simulink model "ACEServoCard"  (R2025b)
settings: Solver=ode4  StartTime=0.0  StopTime=inf  FixedStep=0.01  RelTol=1e-3
undefined symbols (not defined in the file or in its folder): RS422, TTL, UART4, UART5
libraries: simulink x45, etargetslib x26, AFCToolbox x12
settings Model: Creator=zqinghua  LastModifiedBy=zqhkd
settings OptimizationCC: DefaultParameterBehavior=Inlined  EnhancedBackFolding=on  PassReuseOutputArgsAs=Individual arguments  ZeroExternalMemoryAtStartup=off  ZeroInternalMemoryAtStartup=off  OptimizeBlockOrder=speed  DifferentSizesBufferReuse=on  OptimizationCustomize=off  EfficientTunableParamExpr=on
settings DebuggingCC: ParameterTunabilityLossMsg=error
settings HardwareCC: ProdBitPerInt=16.0  ProdBitPerPointer=16.0  ProdBitPerSizeT=16.0  ProdBitPerPtrDiffT=16.0  ProdLargestAtomicFloat=None  ProdWordSize=16.0  ProdHWDeviceType=STMicroelectronics->ST10/Super10
settings SFSimCC: MATLABDynamicMemAlloc=off
settings RTWCC: SystemTargetFile=AFCHawk.tlc  GenCodeOnly=on  TemplateMakefile=ert_default_tmf  GPUComputeCapability=3.5  Description=Embedded Coder
settings CodeAppCC: ForceParamTrailComments=on  IgnoreCustomStorageClasses=off  OperatorAnnotations=on  SimulinkDataObjDesc=on  SFDataObjDesc=on  InsertBlockDesc=on
settings STFCustomTargetCC: SystemTargetFile=AFCHawk.tlc  TargetLangStandard=C99 (ISO)  MultiwordLength=256.0  ModelReferenceCompliant=off  ConcurrentExecutionCompliant=off  CombineOutputUpdateFcns=on  ERTCustomFileBanners=on  SupportContinuousTime=off  SupportNonInlinedSFcns=off  RemoveResetFunc=on  MATLABClassNameForMDSCustomization=Simulink.SoftwareTarget.ERTCustomization  GRTInterface=off  t_DownLoad2Target=on  t_comPort=2.0  t_BuildCPrj2Hex=on  t_comBaud=460800.0
settings ERTTargetCC: ERTCustomFileTemplate=example_file_process.tlc  DynamicArrayContainerType=coder::array  TargetLangStandard=C99 (ISO)  ModelReferenceCompliant=off  ParMdlRefBuildCompliant=off  CompOptLevelCompliant=off  ConcurrentExecutionCompliant=off  ModelStepFunctionPrototypeControlCompliant=off  CPPClassGenCompliant=off  UseToolchainInfoCompliant=off

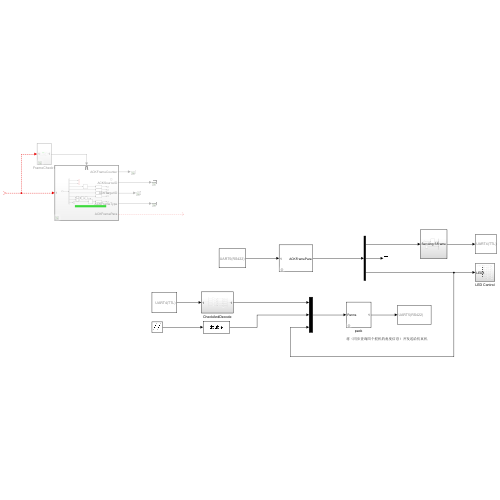
[thumbnail: Simulink's stored preview of the top-level diagram]
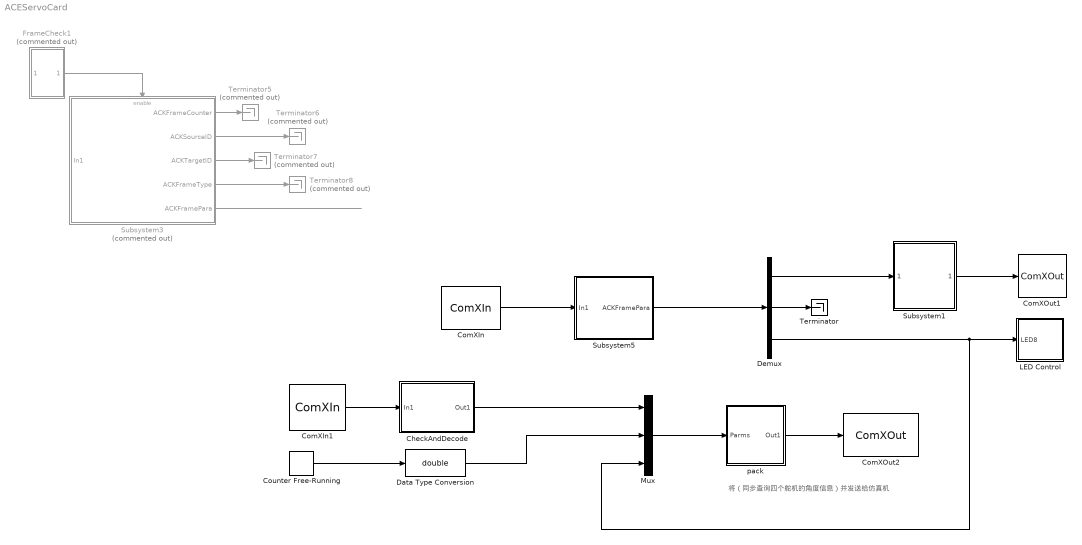
== system ACEServoCard ==
  note: 将（同步查询四个舵机的角度信息）并发送给仿真机
  CheckAndDecode : Subsystem
  ComXIn : AFCToolbox/DeviceModule/ComXIn  Priority=2  g_sampleTime=0.01  g_comPort=UART5(RS422)  g_baudRate=460800  g_dataSize=40  g_parity=0  g_stopBits=1
      settings: SourceProductName=AFCToolbox
  ComXIn1 : AFCToolbox/DeviceModule/ComXIn  Priority=2  g_sampleTime=0.01  g_comPort=UART4(TTL)  g_baudRate=1000000  g_dataSize=4*8  g_parity=0  g_stopBits=1
      settings: SourceProductName=AFCToolbox
  ComXOut1 : AFCToolbox/DeviceModule/ComXOut  Priority=8  g_comPort=UART4(TTL)  g_baudRate=1000000  g_outFreq=1
      settings: SourceProductName=AFCToolbox
  ComXOut2 : AFCToolbox/DeviceModule/ComXOut  Priority=8  g_comPort=UART5(RS422)  g_baudRate=460800  g_outFreq=1
      settings: SourceProductName=AFCToolbox
  Counter Free-Running : simulink/Sources/Counter Free-Running  NumBits=32  tsamp=-1
  Data Type Conversion : DataTypeConversion  OutDataTypeStr=double  SaturateOnIntegerOverflow=off  RndMeth=Floor
  Demux : Demux  Outputs=[4,2,1]
  FrameCheck1 : Subsystem  Commented=on
  LED Control : Subsystem
  Mux : Mux  Inputs=3
  Subsystem1 : Subsystem
  Subsystem3 : Subsystem  Commented=on
  Subsystem5 : Subsystem  mask{length=40, frameType=84}
      mask DialogControl ParameterGroupVar Prompt: 输入字节数
      mask DialogControl Container3 Prompt: 帧类型码(dec)
  Terminator : Terminator
  Terminator{5..8} (4 alike) : Terminator  Commented=on
  pack : Subsystem  mask{frameSender=0, frameType=5}
      mask DialogControl ParameterGroupVar Prompt: 发送方(dec)
      mask DialogControl Container3 Prompt: 帧类型码(dec)
  wires:
  Demux/2 -> Terminator/1
  Demux/1 -> Subsystem1/1(ServAng)
  Demux/3 -> LED Control/1(LED8), Mux/3
  ComXIn1/1 -> CheckAndDecode/1(In1)
  CheckAndDecode/1(Out1) -> Mux/1
  Mux/1 -> pack/1(Parms)
  pack/1(Out1) -> ComXOut2/1
  Subsystem1/1(SFrame) -> ComXOut1/1
  Counter Free-Running/1 -> Data Type Conversion/1
  Data Type Conversion/1 -> Mux/2
  Subsystem3/5(ACKFramePara) -> ?
  ? -> Subsystem3/1(In1), FrameCheck1/1(In1)
  FrameCheck1/1(Out1) -> Subsystem3/Enable
  Subsystem3/4(ACKFrameType) -> Terminator8/1
  Subsystem3/3(ACKTargetID) -> Terminator7/1
  Subsystem3/1(ACKFrameCounter) -> Terminator5/1
  Subsystem3/2(ACKSourceID) -> Terminator6/1
  ComXIn/1 -> Subsystem5/1(In1)
  Subsystem5/1(ACKFramePara) -> Demux/1

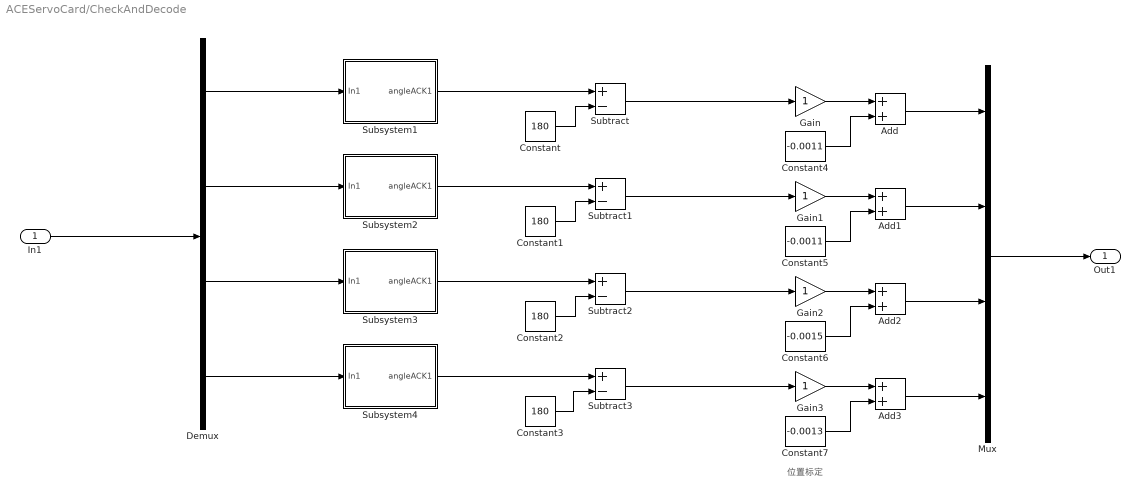
== system ACEServoCard/CheckAndDecode ==
  note: 位置标定
  In1 : Inport
  Add{,1..3} (4 alike) : Sum
  Constant{,1..3} (4 alike) : Constant  Value=180
  Constant4 : Constant  Value=-0.0011
  Constant5 : Constant  Value=-0.0011
  Constant6 : Constant  Value=-0.0015
  Constant7 : Constant  Value=-0.0013
  Demux : Demux  Outputs=[8,8,8,8]
  Gain{,1..3} (4 alike) : Gain
  Mux : Mux
  Subsystem1 : Subsystem
  Subsystem2 : Subsystem
  Subsystem3 : Subsystem
  Subsystem4 : Subsystem
  Subtract{,1..3} (4 alike) : Sum  Inputs=+-
  Out1 : Outport
  wires:
  In1/1 -> Demux/1
  Demux/4 -> Subsystem4/1(In1)
  Demux/3 -> Subsystem3/1(In1)
  Demux/2 -> Subsystem2/1(In1)
  Demux/1 -> Subsystem1/1(In1)
  Subsystem1/1(angleACK1) -> Subtract/1
  Mux/1 -> Out1/1
  Subtract/1 -> Gain/1
  Constant/1 -> Subtract/2
  Constant1/1 -> Subtract1/2
  Subsystem2/1(angleACK1) -> Subtract1/1
  Constant2/1 -> Subtract2/2
  Subsystem3/1(angleACK1) -> Subtract2/1
  Constant3/1 -> Subtract3/2
  Subsystem4/1(angleACK1) -> Subtract3/1
  Constant4/1 -> Add/2
  Gain/1 -> Add/1
  Add/1 -> Mux/1
  Gain1/1 -> Add1/1
  Constant5/1 -> Add1/2
  Subtract1/1 -> Gain1/1
  Subtract2/1 -> Gain2/1
  Constant6/1 -> Add2/2
  Gain2/1 -> Add2/1
  Gain3/1 -> Add3/1
  Constant7/1 -> Add3/2
  Subtract3/1 -> Gain3/1
  Add1/1 -> Mux/2
  Add2/1 -> Mux/3
  Add3/1 -> Mux/4

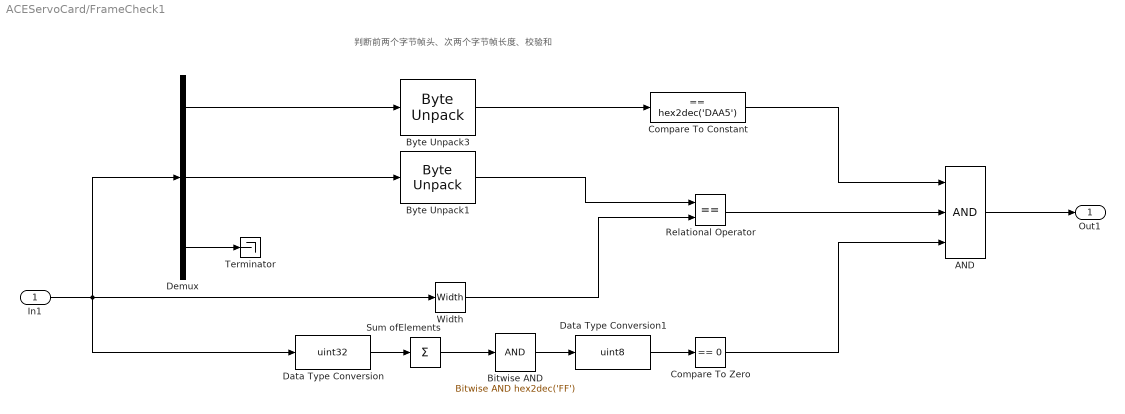
== system ACEServoCard/FrameCheck1 ==
  note: 判断前两个字节帧头、次两个字节帧长度、校验和
  In1 : Inport
  AND : Logic  Inputs=3  IconShape=distinctive  AllPortsSameDT=off  OutDataTypeStr=boolean
  Bitwise AND : simulink/Logic and Bit Operations/Bitwise Operator  logicop=AND  UseBitMask=on  BitMask=hex2dec('FF')  BitMaskRealWorld=Stored Integer
      settings: LibrarySourceBlock=|
      | simulink/Quick Insert/Logic and Bit
      | Operations/Bitwise AND
  Byte Unpack1 : etargetslib/Byte Unpack  dimensions={1}  datatypes={'uint16'}  byteAlign=1
      settings: LibrarySourceBlock=embeddedtargetslib/Host Communication/Byte Unpack
  Byte Unpack3 : etargetslib/Byte Unpack  dimensions={1}  datatypes={'uint16'}  byteAlign=1
      settings: LibrarySourceBlock=embeddedtargetslib/Host Communication/Byte Unpack
  Compare To Constant : simulink/Logic and Bit Operations/Compare To Constant  relop===  const=hex2dec('DAA5')  OutDataTypeStr=boolean
  Compare To Zero : simulink/Logic and Bit Operations/Compare To Zero  relop===  OutDataTypeStr=boolean
  Data Type Conversion : DataTypeConversion  OutDataTypeStr=uint32  SaturateOnIntegerOverflow=off  RndMeth=Floor
  Data Type Conversion1 : DataTypeConversion  OutDataTypeStr=uint8  SaturateOnIntegerOverflow=off  RndMeth=Floor
  Demux : Demux  Outputs=[2,2,-1]
      settings: DisplayOption=none
  Relational Operator : RelationalOperator  Operator===  OutDataTypeStr=boolean  RndMeth=Simplest  InputSameDT=off
  Sum ofElements : Sum  Inputs=+
  Terminator : Terminator
  Width : Width  DataType=uint16
  Out1 : Outport
  wires:
  Sum ofElements/1 -> Bitwise AND/1
  Data Type Conversion1/1 -> Compare To Zero/1
  Demux/3 -> Terminator/1
  Byte Unpack3/1 -> Compare To Constant/1
  Data Type Conversion/1 -> Sum ofElements/1
  In1/1 -> Width/1, Data Type Conversion/1, Demux/1
  Byte Unpack1/1 -> Relational Operator/1
  Demux/2 -> Byte Unpack1/1
  Relational Operator/1 -> AND/2
  Width/1 -> Relational Operator/2
  Compare To Zero/1 -> AND/3
  Compare To Constant/1 -> AND/1
  Demux/1 -> Byte Unpack3/1
  Bitwise AND/1 -> Data Type Conversion1/1
  AND/1 -> Out1/1

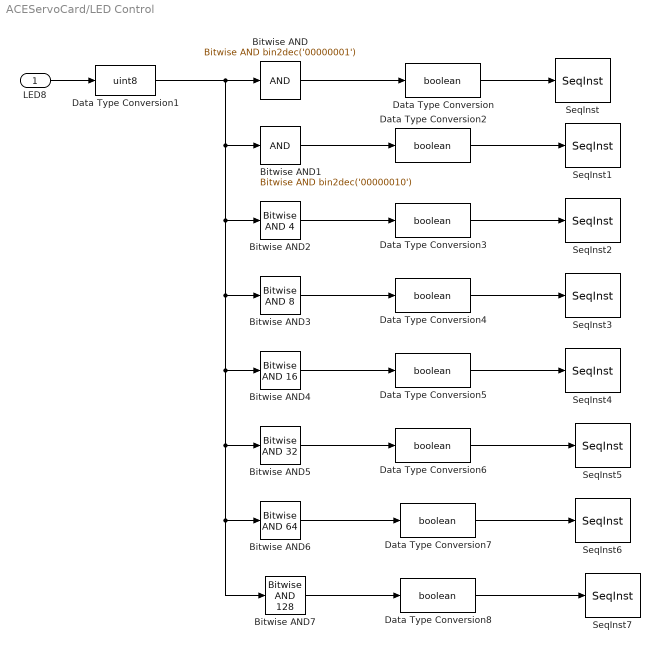
== system ACEServoCard/LED Control ==
  LED8 : Inport
  Bitwise AND : simulink/Logic and Bit Operations/Bitwise Operator  logicop=AND  UseBitMask=on  BitMask=bin2dec('00000001')  BitMaskRealWorld=Stored Integer
      settings: LibrarySourceBlock=|
      | simulink/Quick Insert/Logic and Bit
      | Operations/Bitwise AND
  Bitwise AND1 : simulink/Logic and Bit Operations/Bitwise Operator  logicop=AND  UseBitMask=on  BitMask=bin2dec('00000010')  BitMaskRealWorld=Stored Integer
      settings: LibrarySourceBlock=|
      | simulink/Quick Insert/Logic and Bit
      | Operations/Bitwise AND
  Bitwise AND2 : simulink/Logic and Bit Operations/Bitwise Operator  logicop=AND  UseBitMask=on  BitMask=4  BitMaskRealWorld=Stored Integer
      settings: LibrarySourceBlock=|
      | simulink/Quick Insert/Logic and Bit
      | Operations/Bitwise AND
  Bitwise AND3 : simulink/Logic and Bit Operations/Bitwise Operator  logicop=AND  UseBitMask=on  BitMask=8  BitMaskRealWorld=Stored Integer
      settings: LibrarySourceBlock=|
      | simulink/Quick Insert/Logic and Bit
      | Operations/Bitwise AND
  Bitwise AND4 : simulink/Logic and Bit Operations/Bitwise Operator  logicop=AND  UseBitMask=on  BitMask=16  BitMaskRealWorld=Stored Integer
      settings: LibrarySourceBlock=|
      | simulink/Quick Insert/Logic and Bit
      | Operations/Bitwise AND
  Bitwise AND5 : simulink/Logic and Bit Operations/Bitwise Operator  logicop=AND  UseBitMask=on  BitMask=32  BitMaskRealWorld=Stored Integer
      settings: LibrarySourceBlock=|
      | simulink/Quick Insert/Logic and Bit
      | Operations/Bitwise AND
  Bitwise AND6 : simulink/Logic and Bit Operations/Bitwise Operator  logicop=AND  UseBitMask=on  BitMask=64  BitMaskRealWorld=Stored Integer
      settings: LibrarySourceBlock=|
      | simulink/Quick Insert/Logic and Bit
      | Operations/Bitwise AND
  Bitwise AND7 : simulink/Logic and Bit Operations/Bitwise Operator  logicop=AND  UseBitMask=on  BitMask=128  BitMaskRealWorld=Stored Integer
      settings: LibrarySourceBlock=|
      | simulink/Quick Insert/Logic and Bit
      | Operations/Bitwise AND
  Data Type Conversion{,2..8} (8 alike) : DataTypeConversion  OutDataTypeStr=boolean  SaturateOnIntegerOverflow=off  RndMeth=Floor
  Data Type Conversion1 : DataTypeConversion  OutDataTypeStr=uint8  SaturateOnIntegerOverflow=off  RndMeth=Floor
  SeqInst : AFCToolbox/DeviceModule/SeqInst  Priority=6  g_chanelNo=时序指令1  g_comPort=0  g_instName=0  g_id=0
      settings: SourceProductName=AFCToolbox
  SeqInst1 : AFCToolbox/DeviceModule/SeqInst  Priority=6  g_chanelNo=时序指令2  g_comPort=0  g_instName=0  g_id=0
      settings: SourceProductName=AFCToolbox
  SeqInst2 : AFCToolbox/DeviceModule/SeqInst  Priority=6  g_chanelNo=时序指令3  g_comPort=0  g_instName=0  g_id=0
      settings: SourceProductName=AFCToolbox
  SeqInst3 : AFCToolbox/DeviceModule/SeqInst  Priority=6  g_chanelNo=时序指令4  g_comPort=0  g_instName=0  g_id=0
      settings: SourceProductName=AFCToolbox
  SeqInst4 : AFCToolbox/DeviceModule/SeqInst  Priority=6  g_chanelNo=时序指令5  g_comPort=0  g_instName=0  g_id=0
      settings: SourceProductName=AFCToolbox
  SeqInst5 : AFCToolbox/DeviceModule/SeqInst  Priority=6  g_chanelNo=时序指令6  g_comPort=0  g_instName=0  g_id=0
      settings: SourceProductName=AFCToolbox
  SeqInst6 : AFCToolbox/DeviceModule/SeqInst  Priority=6  g_chanelNo=时序指令7  g_comPort=0  g_instName=0  g_id=0
      settings: SourceProductName=AFCToolbox
  SeqInst7 : AFCToolbox/DeviceModule/SeqInst  Priority=6  g_chanelNo=时序指令8  g_comPort=0  g_instName=0  g_id=0
      settings: SourceProductName=AFCToolbox
  wires:
  Bitwise AND2/1 -> Data Type Conversion3/1
  LED8/1 -> Data Type Conversion1/1
  Bitwise AND5/1 -> Data Type Conversion6/1
  Bitwise AND6/1 -> Data Type Conversion7/1
  Bitwise AND1/1 -> Data Type Conversion2/1
  Bitwise AND3/1 -> Data Type Conversion4/1
  Bitwise AND7/1 -> Data Type Conversion8/1
  Bitwise AND/1 -> Data Type Conversion/1
  Bitwise AND4/1 -> Data Type Conversion5/1
  Data Type Conversion1/1 -> Bitwise AND7/1, Bitwise AND6/1, Bitwise AND5/1, Bitwise AND4/1, Bitwise AND3/1, Bitwise AND2/1, Bitwise AND1/1, Bitwise AND/1
  Data Type Conversion/1 -> SeqInst/1
  Data Type Conversion2/1 -> SeqInst1/1
  Data Type Conversion3/1 -> SeqInst2/1
  Data Type Conversion4/1 -> SeqInst3/1
  Data Type Conversion5/1 -> SeqInst4/1
  Data Type Conversion6/1 -> SeqInst5/1
  Data Type Conversion7/1 -> SeqInst6/1
  Data Type Conversion8/1 -> SeqInst7/1

== system ACEServoCard/Subsystem1 ==
  ServAng : Inport
  Mux : Mux  Inputs=2
  查询四个舵机角度指令 : Subsystem
  设置四个舵机位置与速度指令 : Subsystem
  SFrame : Outport
  wires:
  查询四个舵机角度指令/1(RAng) -> Mux/2
  Mux/1 -> SFrame/1
  设置四个舵机位置与速度指令/1(Frame) -> Mux/1
  ServAng/1 -> 设置四个舵机位置与速度指令/1(Ang)

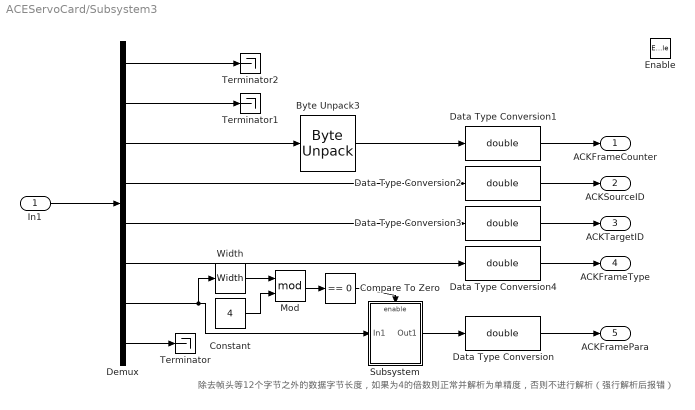
== system ACEServoCard/Subsystem3 ==
  note: 除去帧头等12个字节之外的数据字节长度，如果为4的倍数则正常并解析为单精度，否则不进行解析（强行解析后报错）
  In1 : Inport
  Enable : EnablePort
  Byte Unpack3 : etargetslib/Byte Unpack  dimensions={1}  datatypes={'uint32'}  byteAlign=1
      settings: LibrarySourceBlock=embeddedtargetslib/Host Communication/Byte Unpack
  Compare To Zero : simulink/Logic and Bit Operations/Compare To Zero  relop===  OutDataTypeStr=boolean
  Constant : Constant  Value=4  OutDataTypeStr=uint16
  Data Type Conversion{,1..4} (5 alike) : DataTypeConversion  OutDataTypeStr=double  SaturateOnIntegerOverflow=off  RndMeth=Floor
  Demux : Demux  Outputs=[2,2,4,1,1,1,-1,1]
      settings: DisplayOption=none
  Mod : Math  Operator=mod
  Subsystem : Subsystem
  Terminator : Terminator
  Terminator1 : Terminator
  Terminator2 : Terminator
  Width : Width  DataType=uint16
  ACKFrameCounter : Outport
  ACKSourceID : Outport  Port=2
  ACKTargetID : Outport  Port=3
  ACKFrameType : Outport  Port=4
  ACKFramePara : Outport  Port=5
  wires:
  Compare To Zero/1 -> Subsystem/Enable
  Mod/1 -> Compare To Zero/1
  Data Type Conversion/1 -> ACKFramePara/1
  Subsystem/1(Out1) -> Data Type Conversion/1
  Demux/1 -> Terminator2/1
  Data Type Conversion2/1 -> ACKSourceID/1
  Demux/7 -> Width/1, Subsystem/1(In1)
  Demux/2 -> Terminator1/1
  Demux/5 -> Data Type Conversion3/1
  Demux/6 -> Data Type Conversion4/1
  Data Type Conversion1/1 -> ACKFrameCounter/1
  Data Type Conversion4/1 -> ACKFrameType/1
  Demux/3 -> Byte Unpack3/1
  Byte Unpack3/1 -> Data Type Conversion1/1
  Width/1 -> Mod/1
  Demux/8 -> Terminator/1
  In1/1 -> Demux/1
  Demux/4 -> Data Type Conversion2/1
  Data Type Conversion3/1 -> ACKTargetID/1
  Constant/1 -> Mod/2

== system ACEServoCard/Subsystem5 ==
  In1 : Inport
  FrameCheck1 : Subsystem
  Subsystem1 : Subsystem
  Terminator{1..4} (4 alike) : Terminator
  ACKFramePara : Outport
  wires:
  Subsystem1/4(ACKFrameType) -> Terminator4/1
  Subsystem1/2(ACKSourceID) -> Terminator2/1
  In1/1 -> Subsystem1/1(In1), FrameCheck1/1(In1)
  Subsystem1/1(ACKFrameCounter) -> Terminator1/1  "AFC_ACK_COUNTER"
  FrameCheck1/1(Out1) -> Subsystem1/Enable
  Subsystem1/3(ACKTargetID) -> Terminator3/1
  Subsystem1/5(ACKFramePara) -> ACKFramePara/1

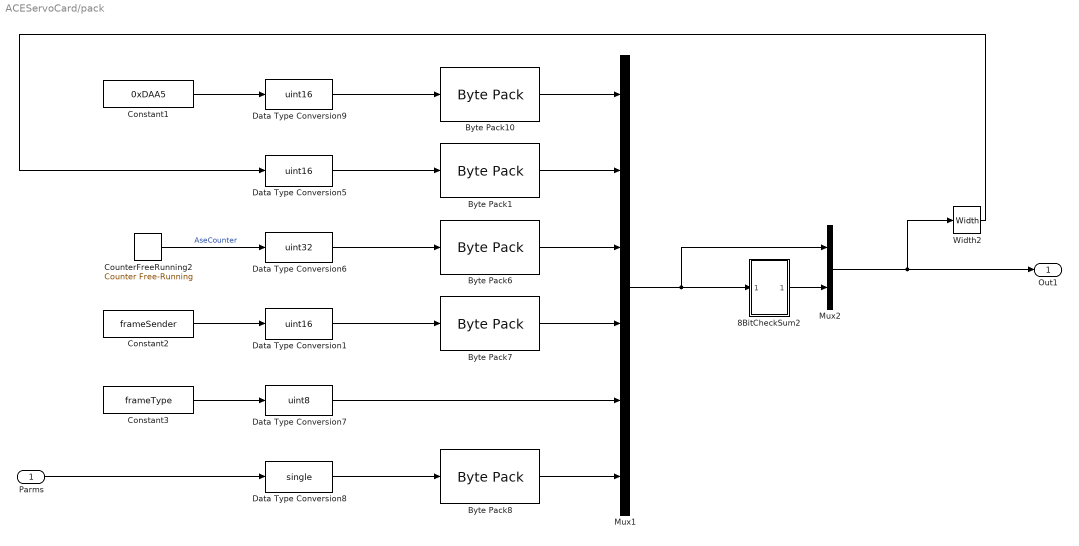
== system ACEServoCard/pack ==
  Parms : Inport
  8BitCheckSum2 : Subsystem
  Byte Pack1 : etargetslib/Byte Pack  datatypes={'uint16'}  byteAlign=1
  Byte Pack10 : etargetslib/Byte Pack  datatypes={'uint16'}  byteAlign=1
  Byte Pack6 : etargetslib/Byte Pack  datatypes={'uint32'}  byteAlign=1
  Byte Pack7 : etargetslib/Byte Pack  datatypes={'uint16'}  byteAlign=1
  Byte Pack8 : etargetslib/Byte Pack  datatypes={'single'}  byteAlign=1
  Constant1 : Constant  Value=0xDAA5
  Constant2 : Constant  Value=frameSender
  Constant3 : Constant  Value=frameType
  CounterFreeRunning2 : simulink/Sources/Counter Free-Running  NumBits=32  tsamp=-1
  Data Type Conversion1 : DataTypeConversion  OutDataTypeStr=uint16  SaturateOnIntegerOverflow=off  RndMeth=Floor
  Data Type Conversion5 : DataTypeConversion  OutDataTypeStr=uint16  SaturateOnIntegerOverflow=off  RndMeth=Floor
  Data Type Conversion6 : DataTypeConversion  OutDataTypeStr=uint32  SaturateOnIntegerOverflow=off  RndMeth=Floor
  Data Type Conversion7 : DataTypeConversion  OutDataTypeStr=uint8  SaturateOnIntegerOverflow=off  RndMeth=Floor
  Data Type Conversion8 : DataTypeConversion  OutDataTypeStr=single  SaturateOnIntegerOverflow=off  RndMeth=Floor
  Data Type Conversion9 : DataTypeConversion  OutDataTypeStr=uint16  SaturateOnIntegerOverflow=off  RndMeth=Floor
  Mux1 : Mux  Inputs=6
  Mux2 : Mux  Inputs=2
  Width2 : Width  DataType=single
  Out1 : Outport
  wires:
  Data Type Conversion6/1 -> Byte Pack6/1
  Data Type Conversion9/1 -> Byte Pack10/1
  Byte Pack6/1 -> Mux1/3
  Mux1/1 -> Mux2/1, 8BitCheckSum2/1(In1)
  Byte Pack8/1 -> Mux1/6
  Data Type Conversion8/1 -> Byte Pack8/1
  8BitCheckSum2/1(Out1) -> Mux2/2
  Byte Pack1/1 -> Mux1/2
  Data Type Conversion1/1 -> Byte Pack7/1
  Byte Pack7/1 -> Mux1/4
  Width2/1 -> Data Type Conversion5/1
  Constant2/1 -> Data Type Conversion1/1
  Byte Pack10/1 -> Mux1/1
  Data Type Conversion7/1 -> Mux1/5
  Constant1/1 -> Data Type Conversion9/1
  CounterFreeRunning2/1 -> Data Type Conversion6/1  "AseCounter"
  Constant3/1 -> Data Type Conversion7/1
  Data Type Conversion5/1 -> Byte Pack1/1
  Parms/1 -> Data Type Conversion8/1
  Mux2/1 -> Out1/1, Width2/1

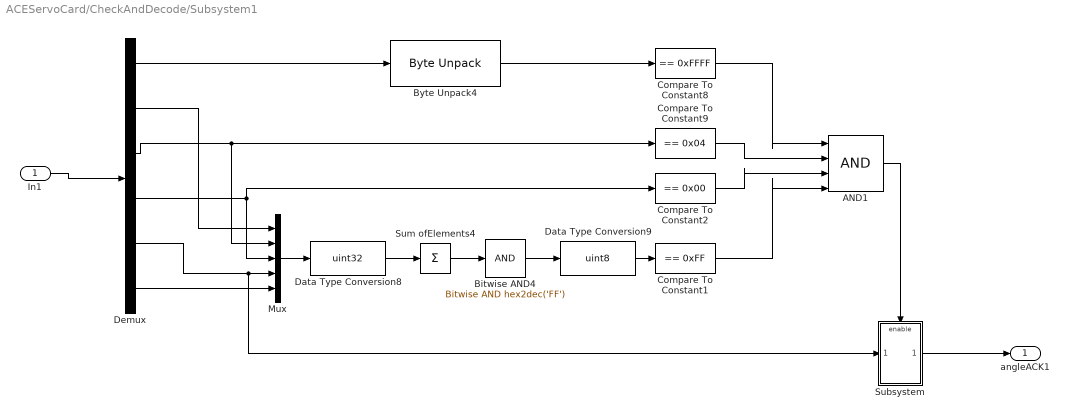
== system ACEServoCard/CheckAndDecode/Subsystem1 ==
  In1 : Inport
  AND1 : Logic  Inputs=4  IconShape=distinctive  AllPortsSameDT=off  OutDataTypeStr=boolean
  Bitwise AND4 : simulink/Logic and Bit Operations/Bitwise Operator  logicop=AND  UseBitMask=on  BitMask=hex2dec('FF')  BitMaskRealWorld=Stored Integer
      settings: LibrarySourceBlock=|
      | simulink/Quick Insert/Logic and Bit
      | Operations/Bitwise AND
  Byte Unpack4 : etargetslib/Byte Unpack  dimensions={[1]}  datatypes={'uint16'}  byteAlign=1
      settings: LibrarySourceBlock=embeddedtargetslib/Host Communication/Byte Unpack
  Compare To Constant1 : simulink/Logic and Bit Operations/Compare To Constant  relop===  const=0xFF  OutDataTypeStr=boolean
  Compare To Constant2 : simulink/Logic and Bit Operations/Compare To Constant  relop===  const=0x00  OutDataTypeStr=boolean
  Compare To Constant8 : simulink/Logic and Bit Operations/Compare To Constant  relop===  const=0xFFFF  OutDataTypeStr=boolean
  Compare To Constant9 : simulink/Logic and Bit Operations/Compare To Constant  relop===  const=0x04  OutDataTypeStr=boolean
  Data Type Conversion8 : DataTypeConversion  OutDataTypeStr=uint32  SaturateOnIntegerOverflow=off  RndMeth=Floor
  Data Type Conversion9 : DataTypeConversion  OutDataTypeStr=uint8  SaturateOnIntegerOverflow=off  RndMeth=Floor
  Demux : Demux  Outputs=[2,1,1,1,2,1]
  Mux : Mux  Inputs=5
  Subsystem : Subsystem
  Sum ofElements4 : Sum  Inputs=+
  angleACK1 : Outport
  wires:
  AND1/1 -> Subsystem/Enable
  Demux/6 -> Mux/5
  Subsystem/1(Outport) -> angleACK1/1
  Demux/5 -> Subsystem/1(In1), Mux/4
  Demux/3 -> Mux/2, Compare To Constant9/1
  Compare To Constant2/1 -> AND1/3
  Demux/2 -> Mux/1
  Data Type Conversion8/1 -> Sum ofElements4/1
  Compare To Constant9/1 -> AND1/2
  Sum ofElements4/1 -> Bitwise AND4/1
  Demux/4 -> Compare To Constant2/1, Mux/3
  Byte Unpack4/1 -> Compare To Constant8/1
  Mux/1 -> Data Type Conversion8/1
  Compare To Constant8/1 -> AND1/1
  Data Type Conversion9/1 -> Compare To Constant1/1
  Bitwise AND4/1 -> Data Type Conversion9/1
  Demux/1 -> Byte Unpack4/1
  Compare To Constant1/1 -> AND1/4
  In1/1 -> Demux/1

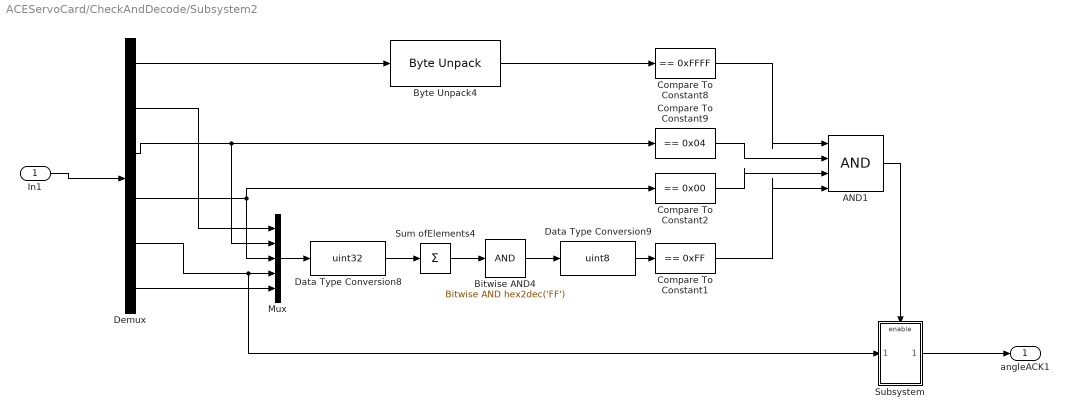
== system ACEServoCard/CheckAndDecode/Subsystem2 ==
  In1 : Inport
  AND1 : Logic  Inputs=4  IconShape=distinctive  AllPortsSameDT=off  OutDataTypeStr=boolean
  Bitwise AND4 : simulink/Logic and Bit Operations/Bitwise Operator  logicop=AND  UseBitMask=on  BitMask=hex2dec('FF')  BitMaskRealWorld=Stored Integer
      settings: LibrarySourceBlock=|
      | simulink/Quick Insert/Logic and Bit
      | Operations/Bitwise AND
  Byte Unpack4 : etargetslib/Byte Unpack  dimensions={[1]}  datatypes={'uint16'}  byteAlign=1
      settings: LibrarySourceBlock=embeddedtargetslib/Host Communication/Byte Unpack
  Compare To Constant1 : simulink/Logic and Bit Operations/Compare To Constant  relop===  const=0xFF  OutDataTypeStr=boolean
  Compare To Constant2 : simulink/Logic and Bit Operations/Compare To Constant  relop===  const=0x00  OutDataTypeStr=boolean
  Compare To Constant8 : simulink/Logic and Bit Operations/Compare To Constant  relop===  const=0xFFFF  OutDataTypeStr=boolean
  Compare To Constant9 : simulink/Logic and Bit Operations/Compare To Constant  relop===  const=0x04  OutDataTypeStr=boolean
  Data Type Conversion8 : DataTypeConversion  OutDataTypeStr=uint32  SaturateOnIntegerOverflow=off  RndMeth=Floor
  Data Type Conversion9 : DataTypeConversion  OutDataTypeStr=uint8  SaturateOnIntegerOverflow=off  RndMeth=Floor
  Demux : Demux  Outputs=[2,1,1,1,2,1]
  Mux : Mux  Inputs=5
  Subsystem : Subsystem
  Sum ofElements4 : Sum  Inputs=+
  angleACK1 : Outport
  wires:
  In1/1 -> Demux/1
  Compare To Constant1/1 -> AND1/4
  Demux/1 -> Byte Unpack4/1
  Bitwise AND4/1 -> Data Type Conversion9/1
  Data Type Conversion9/1 -> Compare To Constant1/1
  Compare To Constant8/1 -> AND1/1
  Mux/1 -> Data Type Conversion8/1
  Byte Unpack4/1 -> Compare To Constant8/1
  Demux/4 -> Mux/3, Compare To Constant2/1
  Sum ofElements4/1 -> Bitwise AND4/1
  Compare To Constant9/1 -> AND1/2
  Data Type Conversion8/1 -> Sum ofElements4/1
  Demux/2 -> Mux/1
  Compare To Constant2/1 -> AND1/3
  Demux/3 -> Compare To Constant9/1, Mux/2
  Demux/5 -> Mux/4, Subsystem/1(In1)
  Subsystem/1(Outport) -> angleACK1/1
  Demux/6 -> Mux/5
  AND1/1 -> Subsystem/Enable

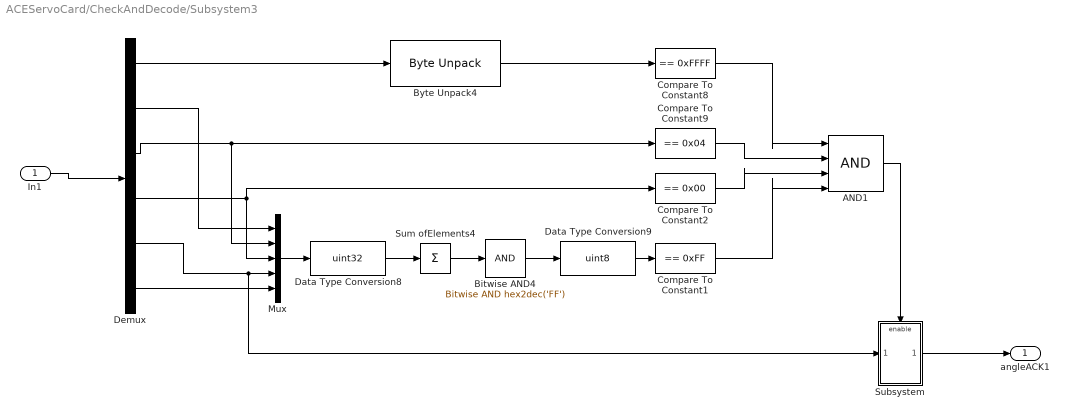
== system ACEServoCard/CheckAndDecode/Subsystem3 ==
  In1 : Inport
  AND1 : Logic  Inputs=4  IconShape=distinctive  AllPortsSameDT=off  OutDataTypeStr=boolean
  Bitwise AND4 : simulink/Logic and Bit Operations/Bitwise Operator  logicop=AND  UseBitMask=on  BitMask=hex2dec('FF')  BitMaskRealWorld=Stored Integer
      settings: LibrarySourceBlock=|
      | simulink/Quick Insert/Logic and Bit
      | Operations/Bitwise AND
  Byte Unpack4 : etargetslib/Byte Unpack  dimensions={[1]}  datatypes={'uint16'}  byteAlign=1
      settings: LibrarySourceBlock=embeddedtargetslib/Host Communication/Byte Unpack
  Compare To Constant1 : simulink/Logic and Bit Operations/Compare To Constant  relop===  const=0xFF  OutDataTypeStr=boolean
  Compare To Constant2 : simulink/Logic and Bit Operations/Compare To Constant  relop===  const=0x00  OutDataTypeStr=boolean
  Compare To Constant8 : simulink/Logic and Bit Operations/Compare To Constant  relop===  const=0xFFFF  OutDataTypeStr=boolean
  Compare To Constant9 : simulink/Logic and Bit Operations/Compare To Constant  relop===  const=0x04  OutDataTypeStr=boolean
  Data Type Conversion8 : DataTypeConversion  OutDataTypeStr=uint32  SaturateOnIntegerOverflow=off  RndMeth=Floor
  Data Type Conversion9 : DataTypeConversion  OutDataTypeStr=uint8  SaturateOnIntegerOverflow=off  RndMeth=Floor
  Demux : Demux  Outputs=[2,1,1,1,2,1]
  Mux : Mux  Inputs=5
  Subsystem : Subsystem
  Sum ofElements4 : Sum  Inputs=+
  angleACK1 : Outport
  wires:
  AND1/1 -> Subsystem/Enable
  Demux/6 -> Mux/5
  Subsystem/1(Outport) -> angleACK1/1
  Demux/5 -> Subsystem/1(In1), Mux/4
  Demux/3 -> Mux/2, Compare To Constant9/1
  Compare To Constant2/1 -> AND1/3
  Demux/2 -> Mux/1
  Data Type Conversion8/1 -> Sum ofElements4/1
  Compare To Constant9/1 -> AND1/2
  Sum ofElements4/1 -> Bitwise AND4/1
  Demux/4 -> Compare To Constant2/1, Mux/3
  Byte Unpack4/1 -> Compare To Constant8/1
  Mux/1 -> Data Type Conversion8/1
  Compare To Constant8/1 -> AND1/1
  Data Type Conversion9/1 -> Compare To Constant1/1
  Bitwise AND4/1 -> Data Type Conversion9/1
  Demux/1 -> Byte Unpack4/1
  Compare To Constant1/1 -> AND1/4
  In1/1 -> Demux/1

== system ACEServoCard/CheckAndDecode/Subsystem4 ==
  In1 : Inport
  AND1 : Logic  Inputs=4  IconShape=distinctive  AllPortsSameDT=off  OutDataTypeStr=boolean
  Bitwise AND4 : simulink/Logic and Bit Operations/Bitwise Operator  logicop=AND  UseBitMask=on  BitMask=hex2dec('FF')  BitMaskRealWorld=Stored Integer
      settings: LibrarySourceBlock=|
      | simulink/Quick Insert/Logic and Bit
      | Operations/Bitwise AND
  Byte Unpack4 : etargetslib/Byte Unpack  dimensions={[1]}  datatypes={'uint16'}  byteAlign=1
      settings: LibrarySourceBlock=embeddedtargetslib/Host Communication/Byte Unpack
  Compare To Constant1 : simulink/Logic and Bit Operations/Compare To Constant  relop===  const=0xFF  OutDataTypeStr=boolean
  Compare To Constant2 : simulink/Logic and Bit Operations/Compare To Constant  relop===  const=0x00  OutDataTypeStr=boolean
  Compare To Constant8 : simulink/Logic and Bit Operations/Compare To Constant  relop===  const=0xFFFF  OutDataTypeStr=boolean
  Compare To Constant9 : simulink/Logic and Bit Operations/Compare To Constant  relop===  const=0x04  OutDataTypeStr=boolean
  Data Type Conversion8 : DataTypeConversion  OutDataTypeStr=uint32  SaturateOnIntegerOverflow=off  RndMeth=Floor
  Data Type Conversion9 : DataTypeConversion  OutDataTypeStr=uint8  SaturateOnIntegerOverflow=off  RndMeth=Floor
  Demux : Demux  Outputs=[2,1,1,1,2,1]
  Mux : Mux  Inputs=5
  Subsystem : Subsystem
  Sum ofElements4 : Sum  Inputs=+
  angleACK1 : Outport
  wires:
  In1/1 -> Demux/1
  Compare To Constant1/1 -> AND1/4
  Demux/1 -> Byte Unpack4/1
  Bitwise AND4/1 -> Data Type Conversion9/1
  Data Type Conversion9/1 -> Compare To Constant1/1
  Compare To Constant8/1 -> AND1/1
  Mux/1 -> Data Type Conversion8/1
  Byte Unpack4/1 -> Compare To Constant8/1
  Demux/4 -> Mux/3, Compare To Constant2/1
  Sum ofElements4/1 -> Bitwise AND4/1
  Compare To Constant9/1 -> AND1/2
  Data Type Conversion8/1 -> Sum ofElements4/1
  Demux/2 -> Mux/1
  Compare To Constant2/1 -> AND1/3
  Demux/3 -> Compare To Constant9/1, Mux/2
  Demux/5 -> Mux/4, Subsystem/1(In1)
  Subsystem/1(Outport) -> angleACK1/1
  Demux/6 -> Mux/5
  AND1/1 -> Subsystem/Enable

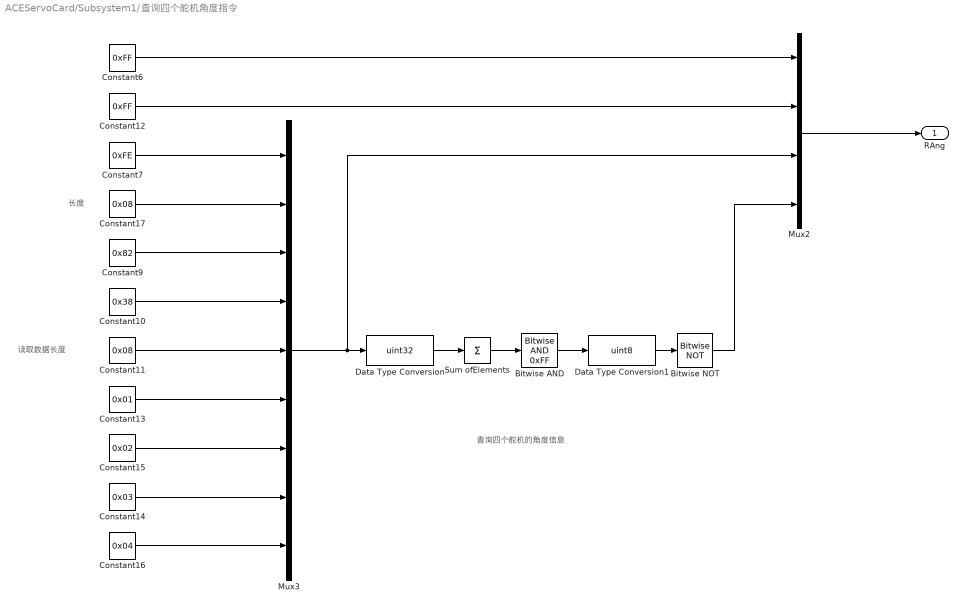
== system ACEServoCard/Subsystem1/查询四个舵机角度指令 ==
  note: 查询四个舵机的角度信息
  note: 长度
  note: 读取数据长度
  Bitwise AND : simulink/Logic and Bit Operations/Bitwise Operator  logicop=AND  UseBitMask=on  BitMask=0xFF  BitMaskRealWorld=Stored Integer
      settings: LibrarySourceBlock=|
      | simulink/Quick Insert/Logic and Bit
      | Operations/Bitwise AND
  Bitwise NOT : simulink/Logic and Bit Operations/Bitwise Operator  logicop=NOT  UseBitMask=off  BitMask=bin2dec('11011001')  BitMaskRealWorld=Stored Integer
      settings: LibrarySourceBlock=|
      | simulink/Quick Insert/Logic and Bit
      | Operations/Bitwise NOT
  Constant10 : Constant  Value=0x38  OutDataTypeStr=uint8
  Constant11 : Constant  Value=0x08  OutDataTypeStr=uint8
  Constant12 : Constant  Value=0xFF  OutDataTypeStr=uint8
  Constant13 : Constant  Value=0x01
  Constant14 : Constant  Value=0x03
  Constant15 : Constant  Value=0x02
  Constant16 : Constant  Value=0x04
  Constant17 : Constant  Value=0x08  OutDataTypeStr=uint8
  Constant6 : Constant  Value=0xFF  OutDataTypeStr=uint8
  Constant7 : Constant  Value=0xFE  OutDataTypeStr=uint8
  Constant9 : Constant  Value=0x82  OutDataTypeStr=uint8
  Data Type Conversion : DataTypeConversion  OutDataTypeStr=uint32  SaturateOnIntegerOverflow=off  RndMeth=Floor
  Data Type Conversion1 : DataTypeConversion  OutDataTypeStr=uint8  SaturateOnIntegerOverflow=off  RndMeth=Floor
  Mux2 : Mux
  Mux3 : Mux  Inputs=9
  Sum ofElements : Sum  Inputs=+
  RAng : Outport
  wires:
  Constant16/1 -> Mux3/9
  Mux3/1 -> Data Type Conversion/1, Mux2/3
  Bitwise AND/1 -> Data Type Conversion1/1
  Data Type Conversion1/1 -> Bitwise NOT/1
  Constant17/1 -> Mux3/2
  Mux2/1 -> RAng/1
  Constant12/1 -> Mux2/2
  Data Type Conversion/1 -> Sum ofElements/1
  Sum ofElements/1 -> Bitwise AND/1
  Constant14/1 -> Mux3/8
  Constant6/1 -> Mux2/1
  Constant13/1 -> Mux3/6
  Constant15/1 -> Mux3/7
  Constant10/1 -> Mux3/4
  Constant11/1 -> Mux3/5
  Bitwise NOT/1 -> Mux2/4
  Constant7/1 -> Mux3/1
  Constant9/1 -> Mux3/3

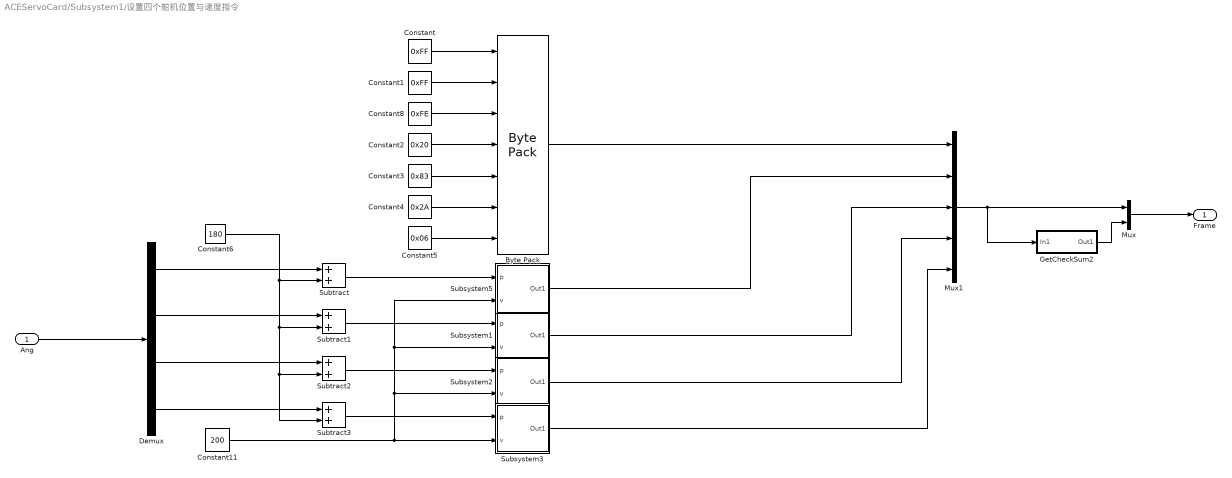
== system ACEServoCard/Subsystem1/设置四个舵机位置与速度指令 ==
  Ang : Inport
  Byte Pack : etargetslib/Byte Pack  datatypes={'uint8','uint8','uint8','uint8','uint8','uint8','uint8'}  byteAlign=1
  Constant : Constant  Value=0xFF  OutDataTypeStr=uint8
  Constant1 : Constant  Value=0xFF  OutDataTypeStr=uint8
  Constant11 : Constant  Value=200
  Constant2 : Constant  Value=0x20  OutDataTypeStr=uint8
  Constant3 : Constant  Value=0x83  OutDataTypeStr=uint8
  Constant4 : Constant  Value=0x2A  OutDataTypeStr=uint8
  Constant5 : Constant  Value=0x06  OutDataTypeStr=uint8
  Constant6 : Constant  Value=180
  Constant8 : Constant  Value=0xFE  OutDataTypeStr=uint8
  Demux : Demux
  GetCheckSum2 : Subsystem
  Mux : Mux  Inputs=2
  Mux1 : Mux  Inputs=5
  Subsystem1 : Subsystem  mask{id=2}
      mask DialogControl ParameterGroupVar Prompt: id
  Subsystem2 : Subsystem  mask{id=3}
      mask DialogControl ParameterGroupVar Prompt: id
  Subsystem3 : Subsystem  mask{id=4}
      mask DialogControl ParameterGroupVar Prompt: id
  Subsystem5 : Subsystem  mask{id=1}
      mask DialogControl ParameterGroupVar Prompt: id
  Subtract{,1..3} (4 alike) : Sum
  Frame : Outport
  wires:
  Mux/1 -> Frame/1
  Constant4/1 -> Byte Pack/6
  Mux1/1 -> Mux/1, GetCheckSum2/1(In1)
  GetCheckSum2/1(Out1) -> Mux/2
  Constant5/1 -> Byte Pack/7
  Constant2/1 -> Byte Pack/4
  Constant1/1 -> Byte Pack/2
  Constant/1 -> Byte Pack/1
  Constant3/1 -> Byte Pack/5
  Constant8/1 -> Byte Pack/3
  Byte Pack/1 -> Mux1/1
  Demux/3 -> Subtract2/1
  Subtract2/1 -> Subsystem2/1(p)
  Subtract3/1 -> Subsystem3/1(p)
  Ang/1 -> Demux/1
  Demux/1 -> Subtract/1
  Constant6/1 -> Subtract3/2, Subtract2/2, Subtract1/2, Subtract/2
  Constant11/1 -> Subsystem3/2(v), Subsystem5/2(v), Subsystem1/2(v), Subsystem2/2(v)
  Subtract1/1 -> Subsystem1/1(p)
  Subtract/1 -> Subsystem5/1(p)
  Demux/2 -> Subtract1/1
  Demux/4 -> Subtract3/1
  Subsystem5/1(Out1) -> Mux1/2
  Subsystem1/1(Out1) -> Mux1/3
  Subsystem2/1(Out1) -> Mux1/4
  Subsystem3/1(Out1) -> Mux1/5

== system ACEServoCard/Subsystem3/Subsystem ==
  In1 : Inport
  Enable : EnablePort
  Byte Unpack1 : etargetslib/Byte Unpack  dimensions={7}  datatypes={'single'}  byteAlign=1
      settings: LibrarySourceBlock=embeddedtargetslib/Host Communication/Byte Unpack
  Out1 : Outport
  wires:
  In1/1 -> Byte Unpack1/1
  Byte Unpack1/1 -> Out1/1

== system ACEServoCard/Subsystem5/FrameCheck1 ==
  note: 判断前两个字节帧头、次1个字节帧长度、校验和
  In1 : Inport
  AND : Logic  Inputs=3  IconShape=distinctive  AllPortsSameDT=off  OutDataTypeStr=boolean
  Bitwise AND : simulink/Logic and Bit Operations/Bitwise Operator  logicop=AND  UseBitMask=on  BitMask=hex2dec('FF')  BitMaskRealWorld=Stored Integer
      settings: LibrarySourceBlock=|
      | simulink/Quick Insert/Logic and Bit
      | Operations/Bitwise AND
  Byte Unpack1 : etargetslib/Byte Unpack  dimensions={1}  datatypes={'uint16'}  byteAlign=1
      settings: LibrarySourceBlock=embeddedtargetslib/Host Communication/Byte Unpack
  Byte Unpack3 : etargetslib/Byte Unpack  dimensions={1}  datatypes={'uint16'}  byteAlign=1
      settings: LibrarySourceBlock=embeddedtargetslib/Host Communication/Byte Unpack
  Compare To Constant : simulink/Logic and Bit Operations/Compare To Constant  relop===  const=0xDAA5  OutDataTypeStr=boolean
  Compare To Zero : simulink/Logic and Bit Operations/Compare To Zero  relop===  OutDataTypeStr=boolean
  Data Type Conversion : DataTypeConversion  OutDataTypeStr=uint32  SaturateOnIntegerOverflow=off  RndMeth=Floor
  Data Type Conversion1 : DataTypeConversion  OutDataTypeStr=uint8  SaturateOnIntegerOverflow=off  RndMeth=Floor
  Demux : Demux  Outputs=[2,2,-1]
      settings: DisplayOption=none
  Relational Operator : RelationalOperator  Operator===  OutDataTypeStr=boolean  RndMeth=Simplest  InputSameDT=off
  Sum ofElements : Sum  Inputs=+
  Terminator : Terminator
  Width : Width  DataType=uint16
  Out1 : Outport
  wires:
  Byte Unpack1/1 -> Relational Operator/1
  Sum ofElements/1 -> Bitwise AND/1
  Data Type Conversion1/1 -> Compare To Zero/1
  Demux/3 -> Terminator/1
  Byte Unpack3/1 -> Compare To Constant/1
  Data Type Conversion/1 -> Sum ofElements/1
  In1/1 -> Width/1, Data Type Conversion/1, Demux/1
  Demux/2 -> Byte Unpack1/1
  Relational Operator/1 -> AND/2
  Width/1 -> Relational Operator/2
  Compare To Zero/1 -> AND/3
  Compare To Constant/1 -> AND/1
  Demux/1 -> Byte Unpack3/1
  Bitwise AND/1 -> Data Type Conversion1/1
  AND/1 -> Out1/1

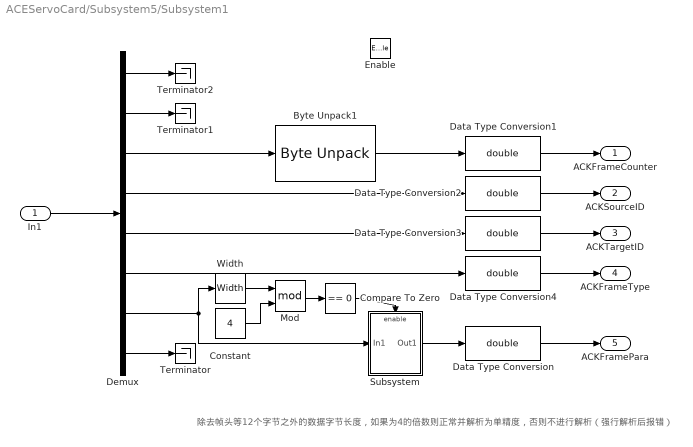
== system ACEServoCard/Subsystem5/Subsystem1 ==
  note: 除去帧头等12个字节之外的数据字节长度，如果为4的倍数则正常并解析为单精度，否则不进行解析（强行解析后报错）
  In1 : Inport
  Enable : EnablePort
  Byte Unpack1 : etargetslib/Byte Unpack  dimensions={1}  datatypes={'uint32'}  byteAlign=1
      settings: LibrarySourceBlock=embeddedtargetslib/Host Communication/Byte Unpack
  Compare To Zero : simulink/Logic and Bit Operations/Compare To Zero  relop===  OutDataTypeStr=boolean
  Constant : Constant  Value=4  OutDataTypeStr=uint16
  Data Type Conversion{,1..4} (5 alike) : DataTypeConversion  OutDataTypeStr=double  SaturateOnIntegerOverflow=off  RndMeth=Floor
  Demux : Demux  Outputs=[2,2,4,1,1,1,-1,1]
      settings: DisplayOption=none
  Mod : Math  Operator=mod
  Subsystem : Subsystem
  Terminator : Terminator
  Terminator1 : Terminator
  Terminator2 : Terminator
  Width : Width  DataType=uint16
  ACKFrameCounter : Outport
  ACKSourceID : Outport  Port=2
  ACKTargetID : Outport  Port=3
  ACKFrameType : Outport  Port=4
  ACKFramePara : Outport  Port=5
  wires:
  Byte Unpack1/1 -> Data Type Conversion1/1
  Compare To Zero/1 -> Subsystem/Enable
  Mod/1 -> Compare To Zero/1
  Data Type Conversion/1 -> ACKFramePara/1
  Demux/1 -> Terminator2/1
  Data Type Conversion2/1 -> ACKSourceID/1
  Demux/7 -> Width/1, Subsystem/1(In1)
  Demux/2 -> Terminator1/1
  Demux/5 -> Data Type Conversion3/1
  Demux/6 -> Data Type Conversion4/1
  Data Type Conversion1/1 -> ACKFrameCounter/1
  Data Type Conversion4/1 -> ACKFrameType/1
  Demux/3 -> Byte Unpack1/1
  Width/1 -> Mod/1
  Demux/8 -> Terminator/1
  In1/1 -> Demux/1
  Demux/4 -> Data Type Conversion2/1
  Data Type Conversion3/1 -> ACKTargetID/1
  Constant/1 -> Mod/2
  Subsystem/1(Out1) -> Data Type Conversion/1

== system ACEServoCard/pack/8BitCheckSum2 ==
  In1 : Inport
  Add : Sum
  Bitwise AND : simulink/Logic and Bit Operations/Bitwise Operator  logicop=AND  UseBitMask=on  BitMask=hex2dec('FF')  BitMaskRealWorld=Stored Integer
      settings: LibrarySourceBlock=|
      | simulink/Quick Insert/Logic and Bit
      | Operations/Bitwise AND
  Bitwise AND1 : simulink/Logic and Bit Operations/Bitwise Operator  logicop=AND  UseBitMask=on  BitMask=hex2dec('FF')  BitMaskRealWorld=Stored Integer
      settings: LibrarySourceBlock=|
      | simulink/Quick Insert/Logic and Bit
      | Operations/Bitwise AND
  Bitwise NOT : simulink/Logic and Bit Operations/Bitwise Operator  logicop=NOT  UseBitMask=off  BitMask=bin2dec('11011001')  BitMaskRealWorld=Stored Integer
      settings: LibrarySourceBlock=|
      | simulink/Quick Insert/Logic and Bit
      | Operations/Bitwise NOT
  Constant5 : Constant
  Data Type Conversion10 : DataTypeConversion  OutDataTypeStr=uint8  SaturateOnIntegerOverflow=off  RndMeth=Floor
  Data Type Conversion11 : DataTypeConversion  OutDataTypeStr=uint16  SaturateOnIntegerOverflow=off  RndMeth=Floor
  Data Type Conversion12 : DataTypeConversion  OutDataTypeStr=uint8  SaturateOnIntegerOverflow=off  RndMeth=Floor
  Data Type Conversion8 : DataTypeConversion  OutDataTypeStr=uint32  SaturateOnIntegerOverflow=off  RndMeth=Floor
  Data Type Conversion9 : DataTypeConversion  OutDataTypeStr=uint16  SaturateOnIntegerOverflow=off  RndMeth=Floor
  Sum of Elements : Sum  Inputs=+
  Out1 : Outport
  wires:
  Bitwise NOT/1 -> Data Type Conversion9/1
  Constant5/1 -> Data Type Conversion11/1
  Sum of Elements/1 -> Bitwise AND/1
  Bitwise AND/1 -> Data Type Conversion10/1
  Add/1 -> Bitwise AND1/1
  Data Type Conversion9/1 -> Add/1
  Data Type Conversion11/1 -> Add/2
  Data Type Conversion8/1 -> Sum of Elements/1
  Data Type Conversion10/1 -> Bitwise NOT/1
  In1/1 -> Data Type Conversion8/1
  Data Type Conversion12/1 -> Out1/1
  Bitwise AND1/1 -> Data Type Conversion12/1

== system ACEServoCard/CheckAndDecode/Subsystem1/Subsystem ==
  In1 : Inport
  Enable : EnablePort
  Byte Unpack22 : etargetslib/Byte Unpack  dimensions={[1]}  datatypes={'int16'}  byteAlign=1
      settings: LibrarySourceBlock=embeddedtargetslib/Host Communication/Byte Unpack
  Constant23 : Constant  Value=360/4096
  Data Type Conversion2 : DataTypeConversion  OutDataTypeStr=double  SaturateOnIntegerOverflow=off  RndMeth=Floor
  Divide24 : Product  Inputs=**
  Outport : Outport
  wires:
  Data Type Conversion2/1 -> Divide24/2
  In1/1 -> Byte Unpack22/1
  Constant23/1 -> Divide24/1
  Byte Unpack22/1 -> Data Type Conversion2/1
  Divide24/1 -> Outport/1

== system ACEServoCard/CheckAndDecode/Subsystem2/Subsystem ==
  In1 : Inport
  Enable : EnablePort
  Byte Unpack22 : etargetslib/Byte Unpack  dimensions={[1]}  datatypes={'int16'}  byteAlign=1
      settings: LibrarySourceBlock=embeddedtargetslib/Host Communication/Byte Unpack
  Constant23 : Constant  Value=360/4096
  Data Type Conversion2 : DataTypeConversion  OutDataTypeStr=double  SaturateOnIntegerOverflow=off  RndMeth=Floor
  Divide24 : Product  Inputs=**
  Outport : Outport
  wires:
  Divide24/1 -> Outport/1
  Byte Unpack22/1 -> Data Type Conversion2/1
  Constant23/1 -> Divide24/1
  In1/1 -> Byte Unpack22/1
  Data Type Conversion2/1 -> Divide24/2

== system ACEServoCard/CheckAndDecode/Subsystem3/Subsystem ==
  In1 : Inport
  Enable : EnablePort
  Byte Unpack22 : etargetslib/Byte Unpack  dimensions={[1]}  datatypes={'int16'}  byteAlign=1
      settings: LibrarySourceBlock=embeddedtargetslib/Host Communication/Byte Unpack
  Constant23 : Constant  Value=360/4096
  Data Type Conversion2 : DataTypeConversion  OutDataTypeStr=double  SaturateOnIntegerOverflow=off  RndMeth=Floor
  Divide24 : Product  Inputs=**
  Outport : Outport
  wires:
  Data Type Conversion2/1 -> Divide24/2
  In1/1 -> Byte Unpack22/1
  Constant23/1 -> Divide24/1
  Byte Unpack22/1 -> Data Type Conversion2/1
  Divide24/1 -> Outport/1

== system ACEServoCard/CheckAndDecode/Subsystem4/Subsystem ==
  In1 : Inport
  Enable : EnablePort
  Byte Unpack22 : etargetslib/Byte Unpack  dimensions={[1]}  datatypes={'int16'}  byteAlign=1
      settings: LibrarySourceBlock=embeddedtargetslib/Host Communication/Byte Unpack
  Constant23 : Constant  Value=360/4096
  Data Type Conversion2 : DataTypeConversion  OutDataTypeStr=double  SaturateOnIntegerOverflow=off  RndMeth=Floor
  Divide24 : Product  Inputs=**
  Outport : Outport
  wires:
  Divide24/1 -> Outport/1
  Byte Unpack22/1 -> Data Type Conversion2/1
  Constant23/1 -> Divide24/1
  In1/1 -> Byte Unpack22/1
  Data Type Conversion2/1 -> Divide24/2

== system ACEServoCard/Subsystem1/设置四个舵机位置与速度指令/GetCheckSum2 ==
  In1 : Inport
  Bitwise AND4 : simulink/Logic and Bit Operations/Bitwise Operator  logicop=AND  UseBitMask=on  BitMask=hex2dec('FF')  BitMaskRealWorld=Stored Integer
      settings: LibrarySourceBlock=|
      | simulink/Quick Insert/Logic and Bit
      | Operations/Bitwise AND
  Bitwise NOT : simulink/Logic and Bit Operations/Bitwise Operator  logicop=NOT  UseBitMask=off  BitMask=bin2dec('11011001')  BitMaskRealWorld=Stored Integer
      settings: LibrarySourceBlock=|
      | simulink/Quick Insert/Logic and Bit
      | Operations/Bitwise NOT
  Data Type Conversion8 : DataTypeConversion  OutDataTypeStr=uint32  SaturateOnIntegerOverflow=off  RndMeth=Floor
  Data Type Conversion9 : DataTypeConversion  OutDataTypeStr=uint8  SaturateOnIntegerOverflow=off  RndMeth=Floor
  Demux1 : Demux  Outputs=[2,-1]
  Sum ofElements4 : Sum  Inputs=+
  Terminator : Terminator
  Out1 : Outport
  wires:
  Data Type Conversion9/1 -> Bitwise NOT/1
  Data Type Conversion8/1 -> Sum ofElements4/1
  Sum ofElements4/1 -> Bitwise AND4/1
  Bitwise AND4/1 -> Data Type Conversion9/1
  Demux1/2 -> Data Type Conversion8/1
  Demux1/1 -> Terminator/1
  In1/1 -> Demux1/1
  Bitwise NOT/1 -> Out1/1

== system ACEServoCard/Subsystem1/设置四个舵机位置与速度指令/Subsystem1 ==
  p : Inport
  v : Inport  Port=2
  Byte Pack : etargetslib/Byte Pack  datatypes={'uint8','uint16','uint16','uint16'}  byteAlign=1
  Constant : Constant  Value=id
  Constant2 : Constant  Value=4096/60  OutDataTypeStr=double
  Constant3 : Constant  Value=360/4096  OutDataTypeStr=double
  Data Type Conversion4 : DataTypeConversion  OutDataTypeStr=uint16  SaturateOnIntegerOverflow=off  RndMeth=Floor
  Data Type Conversion5 : DataTypeConversion  OutDataTypeStr=uint8  SaturateOnIntegerOverflow=off  RndMeth=Floor
  Data Type Conversion6 : DataTypeConversion  OutDataTypeStr=uint16  SaturateOnIntegerOverflow=off  RndMeth=Floor
  Divide3 : Product  Inputs=*/
  Divide4 : Product  Inputs=**
  time : Constant  Value=0  OutDataTypeStr=uint16
  Out1 : Outport
  wires:
  Byte Pack/1 -> Out1/1
  Constant/1 -> Data Type Conversion5/1
  p/1 -> Divide3/1
  Data Type Conversion5/1 -> Byte Pack/1
  v/1 -> Divide4/1
  time/1 -> Byte Pack/3
  Divide4/1 -> Data Type Conversion6/1
  Data Type Conversion4/1 -> Byte Pack/2
  Constant3/1 -> Divide3/2
  Constant2/1 -> Divide4/2
  Data Type Conversion6/1 -> Byte Pack/4
  Divide3/1 -> Data Type Conversion4/1

== system ACEServoCard/Subsystem1/设置四个舵机位置与速度指令/Subsystem2 ==
  p : Inport
  v : Inport  Port=2
  Byte Pack : etargetslib/Byte Pack  datatypes={'uint8','uint16','uint16','uint16'}  byteAlign=1
  Constant : Constant  Value=id
  Constant2 : Constant  Value=4096/60  OutDataTypeStr=double
  Constant3 : Constant  Value=360/4096  OutDataTypeStr=double
  Data Type Conversion4 : DataTypeConversion  OutDataTypeStr=uint16  SaturateOnIntegerOverflow=off  RndMeth=Floor
  Data Type Conversion5 : DataTypeConversion  OutDataTypeStr=uint8  SaturateOnIntegerOverflow=off  RndMeth=Floor
  Data Type Conversion6 : DataTypeConversion  OutDataTypeStr=uint16  SaturateOnIntegerOverflow=off  RndMeth=Floor
  Divide3 : Product  Inputs=*/
  Divide4 : Product  Inputs=**
  time : Constant  Value=0  OutDataTypeStr=uint16
  Out1 : Outport
  wires:
  Divide3/1 -> Data Type Conversion4/1
  Data Type Conversion6/1 -> Byte Pack/4
  Constant2/1 -> Divide4/2
  Constant3/1 -> Divide3/2
  Data Type Conversion4/1 -> Byte Pack/2
  Divide4/1 -> Data Type Conversion6/1
  time/1 -> Byte Pack/3
  v/1 -> Divide4/1
  Data Type Conversion5/1 -> Byte Pack/1
  p/1 -> Divide3/1
  Constant/1 -> Data Type Conversion5/1
  Byte Pack/1 -> Out1/1

== system ACEServoCard/Subsystem1/设置四个舵机位置与速度指令/Subsystem3 ==
  p : Inport
  v : Inport  Port=2
  Byte Pack : etargetslib/Byte Pack  datatypes={'uint8','uint16','uint16','uint16'}  byteAlign=1
  Constant : Constant  Value=id
  Constant2 : Constant  Value=4096/60  OutDataTypeStr=double
  Constant3 : Constant  Value=360/4096  OutDataTypeStr=double
  Data Type Conversion4 : DataTypeConversion  OutDataTypeStr=uint16  SaturateOnIntegerOverflow=off  RndMeth=Floor
  Data Type Conversion5 : DataTypeConversion  OutDataTypeStr=uint8  SaturateOnIntegerOverflow=off  RndMeth=Floor
  Data Type Conversion6 : DataTypeConversion  OutDataTypeStr=uint16  SaturateOnIntegerOverflow=off  RndMeth=Floor
  Divide3 : Product  Inputs=*/
  Divide4 : Product  Inputs=**
  time : Constant  Value=0  OutDataTypeStr=uint16
  Out1 : Outport
  wires:
  Byte Pack/1 -> Out1/1
  Constant/1 -> Data Type Conversion5/1
  p/1 -> Divide3/1
  Data Type Conversion5/1 -> Byte Pack/1
  v/1 -> Divide4/1
  time/1 -> Byte Pack/3
  Divide4/1 -> Data Type Conversion6/1
  Data Type Conversion4/1 -> Byte Pack/2
  Constant3/1 -> Divide3/2
  Constant2/1 -> Divide4/2
  Data Type Conversion6/1 -> Byte Pack/4
  Divide3/1 -> Data Type Conversion4/1

== system ACEServoCard/Subsystem1/设置四个舵机位置与速度指令/Subsystem5 ==
  p : Inport
  v : Inport  Port=2
  Byte Pack : etargetslib/Byte Pack  datatypes={'uint8','uint16','uint16','uint16'}  byteAlign=1
  Constant : Constant  Value=id
  Constant2 : Constant  Value=4096/60  OutDataTypeStr=double
  Constant3 : Constant  Value=360/4096  OutDataTypeStr=double
  Data Type Conversion4 : DataTypeConversion  OutDataTypeStr=uint16  SaturateOnIntegerOverflow=off  RndMeth=Floor
  Data Type Conversion5 : DataTypeConversion  OutDataTypeStr=uint8  SaturateOnIntegerOverflow=off  RndMeth=Floor
  Data Type Conversion6 : DataTypeConversion  OutDataTypeStr=uint16  SaturateOnIntegerOverflow=off  RndMeth=Floor
  Divide3 : Product  Inputs=*/
  Divide4 : Product  Inputs=**
  time : Constant  Value=0  OutDataTypeStr=uint16
  Out1 : Outport
  wires:
  Divide3/1 -> Data Type Conversion4/1
  Data Type Conversion6/1 -> Byte Pack/4
  Constant2/1 -> Divide4/2
  Constant3/1 -> Divide3/2
  Data Type Conversion4/1 -> Byte Pack/2
  Divide4/1 -> Data Type Conversion6/1
  time/1 -> Byte Pack/3
  v/1 -> Divide4/1
  Data Type Conversion5/1 -> Byte Pack/1
  p/1 -> Divide3/1
  Constant/1 -> Data Type Conversion5/1
  Byte Pack/1 -> Out1/1

== system ACEServoCard/Subsystem5/Subsystem1/Subsystem ==
  In1 : Inport
  Enable : EnablePort
  Byte Unpack1 : etargetslib/Byte Unpack  dimensions={(length-12)/4}  datatypes={'single'}  byteAlign=1
      settings: LibrarySourceBlock=embeddedtargetslib/Host Communication/Byte Unpack
  Out1 : Outport
  wires:
  Byte Unpack1/1 -> Out1/1
  In1/1 -> Byte Unpack1/1
